simulink subsystem "StudentTemplate_MTMTAD006_M1"  (R2025a)
settings: Solver=VariableStepAuto  StartTime=0.0  StopTime=10.0  RelTol=1e-3
libraries: eeGeneralControl x3, simulink x2, slpidlib x1, cstblocks x1, dspstat3 x1
settings Model: Creator=JesseJabezArendse  LastModifiedBy=MTMTAD006

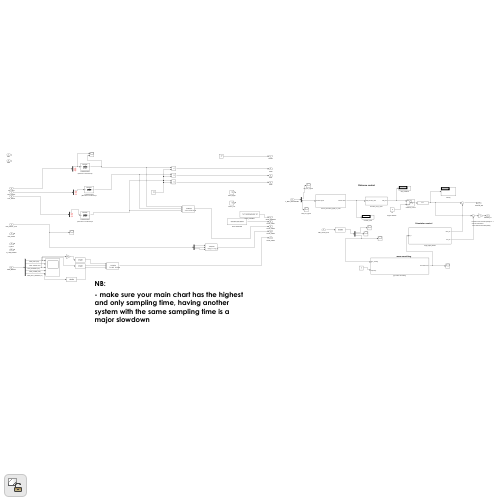
[thumbnail: Simulink's stored preview of the top-level diagram]
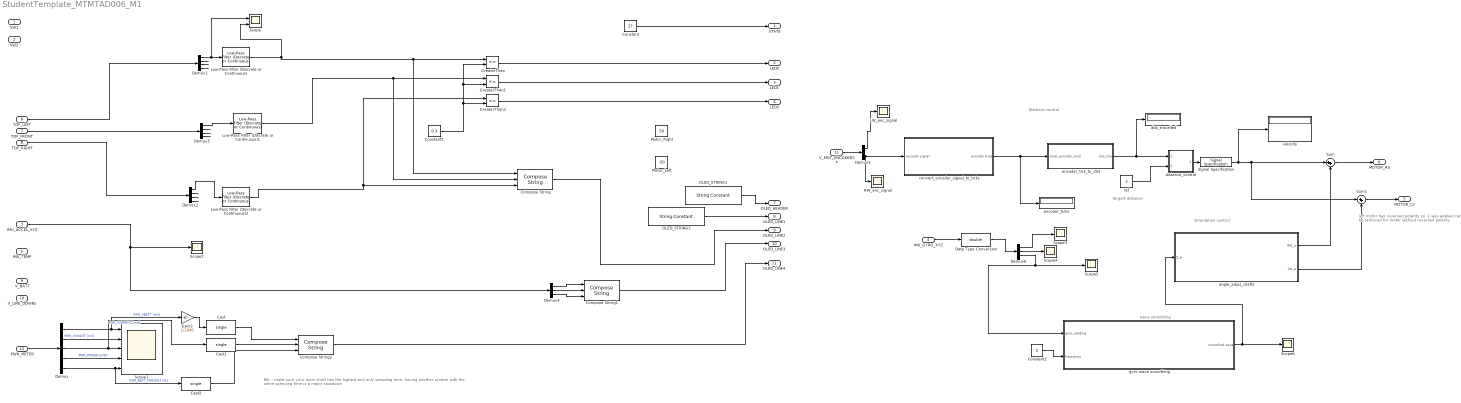
== system StudentTemplate_MTMTAD006_M1 ==
  note: left motor has reversed polarity so -1 was applied
      | can be removed for
      |  motor without reversed polarity
  note: targert distance
  note: wave smoothing
  note: Orientation control
  note: Distance control
  note: NB:
      |
      | - make sure your main chart has the highest and only sampling time, having another system with the same sampling time is a major slowdown
  SW1 : Inport
  SW2 : Inport  Port=2
  IMU_ACCEL_XYZ : Inport  Port=3
  IMU_GYRO_XYZ : Inport  Port=4
  IMU_TEMP : Inport  Port=5
  TOF_LEFT : Inport  Port=6
  TOF_FRONT : Inport  Port=7
  TOF_RIGHT : Inport  Port=8
  V_BATT : Inport  Port=9
  V_LINE_DOWNs : Inport  Port=10
  V_MOT_ENCODERSs : Inport  Port=11
  PWR_METER : Inport  Port=12
  Cast : DataTypeConversion  OutDataTypeStr=single  SaturateOnIntegerOverflow=off  RndMeth=Floor
  Cast1 : DataTypeConversion  OutDataTypeStr=single  SaturateOnIntegerOverflow=off  RndMeth=Floor
  Cast2 : DataTypeConversion  OutDataTypeStr=single  SaturateOnIntegerOverflow=off  RndMeth=Floor
  Compose String : ComposeString  Format="\"L%1.2f F%1.2f R%1.2f\""
  Compose String1 : ComposeString  Format="\"X%2.1f  Y%2.1f  Z%2.1f\""
  Compose String2 : ComposeString  Format="\"%1.2fV  %3.0fmA  %2.0f%%\""
  Constant : Constant  Value=27
  Constant1 : Constant  Value=0.3  SampleTime=-1
  Constant2 : Constant  Value=5
  Data Type Conversion : DataTypeConversion  OutDataTypeStr=double  SaturateOnIntegerOverflow=off  RndMeth=Floor
  Demux : Demux  Outputs=5
  Demux1 : Demux
  Demux2 : Demux
  Demux3 : Demux
  Demux4 : Demux  Outputs=3
  Demux5 : Demux  Outputs=2
  Demux6 : Demux  Outputs=3
  Gain2 : Gain  Gain=1/1000
  GreaterThan : RelationalOperator  Operator=<=  OutDataTypeStr=boolean  RndMeth=Simplest  InputSameDT=off
  GreaterThan1 : RelationalOperator  Operator=<=  OutDataTypeStr=boolean  RndMeth=Simplest  InputSameDT=off
  GreaterThan2 : RelationalOperator  Operator=<=  OutDataTypeStr=boolean  RndMeth=Simplest  InputSameDT=off
  LW_enc_signal : Scope
      settings: ActiveDisplayYMinimum=0.18771853517235504  ActiveDisplayYMaximum=0.24579643082508262  DataLoggingVariableName=ScopeData3
  Low-Pass Filter (Discrete or Continuous) : eeGeneralControl/Low-Pass Filter (Discrete or Continuous)  K=1  T=0.1  B=inf  A=-inf  init_option=Inherited from block input  x0=0  Ts=-1
  Low-Pass Filter (Discrete or Continuous)1 : eeGeneralControl/Low-Pass Filter (Discrete or Continuous)  K=1  T=0.1  B=inf  A=-inf  init_option=Inherited from block input  x0=0  Ts=-1
  Low-Pass Filter (Discrete or Continuous)2 : eeGeneralControl/Low-Pass Filter (Discrete or Continuous)  K=1  T=0.1  B=inf  A=-inf  init_option=Inherited from block input  x0=0  Ts=-1
  Motor_Left : Constant  Value=-50
  Motor_Right : Constant  Value=50
  OLED_STRING1 : StringConstant  String="\"UCT MICROMOUSE '25\""
  OLED_STRING2 : StringConstant  String="\"Simulink Data Demo\""
  RW_enc_signal : Scope
      settings: ActiveDisplayYMinimum=-0.18879534928548519  ActiveDisplayYMaximum=0.86303657781243615  DataLoggingVariableName=ScopeData4
  Scope : Scope  NumInputPorts=2
      settings: ActiveDisplayYMinimum=0.22759  ActiveDisplayYMaximum=0.52326  DataLoggingVariableName=ScopeData7
  Scope1 : Scope  NumInputPorts=5
      settings: ActiveDisplayYMinimum=-437.5  ActiveDisplayYMaximum=3937.5  DataLoggingVariableName=ScopeData6
  Scope{2..6} (5 alike) : Scope
      Scope2 settings: DataLoggingVariableName=ScopeData5
      Scope3 settings: ActiveDisplayYMinimum=-6.6655610351062915  ActiveDisplayYMaximum=8.47328179489563
      Scope4 settings: ActiveDisplayYMinimum=-9.9323014882304754  ActiveDisplayYMaximum=8.7797280520113681  DataLoggingVariableName=ScopeData10
      Scope5 settings: ActiveDisplayYMinimum=-4.0435245770175019  ActiveDisplayYMaximum=1.9742402712877856  DataLoggingVariableName=ScopeData9
      Scope6 settings: ActiveDisplayYMinimum=-2.7558239104233082  ActiveDisplayYMaximum=4.258969164786496  DataLoggingVariableName=ScopeData11
  Signal Specification : SignalSpecification  Dimensions=1
  Sum : Sum  Inputs=|++
  Sum1 : Sum  Inputs=|++
  angle_adjus_draft2 : Subsystem
  convert_encoder_signal_to_ticks : Subsystem
  dist_travelled : Display
  distance_control : Stateflow chart  TreatAsAtomicUnit=on
  encoder_tick_to_dist : Subsystem
  encoder_ticks : Display
  "gyro wave smoothing " : Subsystem
  ref : Constant  Value=2
  velocity : Display
  STATE : Outport
  LED0 : Outport  Port=2
  LED1 : Outport  Port=3
  LED2 : Outport  Port=4
  MOTOR_LS : Outport  Port=5
  MOTOR_RS : Outport  Port=6
  OLED_HEADER : Outport  Port=7
  OLED_LINE1 : Outport  Port=8
  OLED_LINE2 : Outport  Port=9
  OLED_LINE3 : Outport  Port=10
  OLED_LINE4 : Outport  Port=11
  wires:
  TOF_FRONT/1 -> Demux3/1
  OLED_STRING2/1 -> OLED_LINE1/1
  Demux2/1 -> Low-Pass Filter (Discrete or Continuous)2/1
  Demux2/3 -> ?
  Demux2/2 -> ?
  Demux2/4 -> ?
  Compose String1/1 -> OLED_LINE3/1
  Low-Pass Filter (Discrete or Continuous)1/1 -> Compose String/2, GreaterThan1/1
  GreaterThan1/1 -> LED1/1
  Demux3/3 -> ?
  TOF_RIGHT/1 -> Demux2/1
  Demux3/4 -> ?
  Demux3/2 -> ?
  Demux1/2 -> ?
  Demux3/1 -> Low-Pass Filter (Discrete or Continuous)1/1
  OLED_STRING1/1 -> OLED_HEADER/1
  Demux1/1 -> Scope/1, Low-Pass Filter (Discrete or Continuous)/1
  Compose String/1 -> OLED_LINE2/1
  Constant1/1 -> GreaterThan2/2, GreaterThan1/2, GreaterThan/2
  Demux1/4 -> ?
  GreaterThan2/1 -> LED2/1
  TOF_LEFT/1 -> Demux1/1
  GreaterThan/1 -> LED0/1
  Demux1/3 -> ?
  PWR_METER/1 -> Demux/1
  Demux/1 -> Scope1/1, Gain2/1  "PWR_VBATT [mV]"
  Demux/2 -> Scope1/2  "PWR_VSHUNT [mV]"
  Demux/3 -> Scope1/3, Cast1/1  "PWR_CURRENT [mA]"
  Demux/4 -> Scope1/4  "PWR_POWER [mW]"
  Demux/5 -> Scope1/5, Cast2/1  "PWR_BATT_PERCENT [%]"
  IMU_ACCEL_XYZ/1 -> Demux4/1, Scope2/1
  Demux4/1 -> Compose String1/1
  Demux4/2 -> Compose String1/2
  Demux4/3 -> Compose String1/3
  Compose String2/1 -> OLED_LINE4/1
  Gain2/1 -> Cast/1
  Cast/1 -> Compose String2/1
  Cast1/1 -> Compose String2/2
  Cast2/1 -> Compose String2/3
  Low-Pass Filter (Discrete or Continuous)2/1 -> Compose String/3, GreaterThan2/1
  Low-Pass Filter (Discrete or Continuous)/1 -> Scope/2, Compose String/1, GreaterThan/1
  Constant/1 -> STATE/1
  Demux5/2 -> convert_encoder_signal_to_ticks/1(encoder signal), RW_enc_signal/1
  Demux5/1 -> LW_enc_signal/1
  V_MOT_ENCODERSs/1 -> Demux5/1
  Signal Specification/1 -> Sum/1, Sum1/1, velocity/1
  distance_control/1(ang_vel) -> Signal Specification/1
  ref/1 -> distance_control/2(target)
  convert_encoder_signal_to_ticks/1(encoder ticks) -> encoder_tick_to_dist/1(total_encoder_ticks), encoder_ticks/1
  encoder_tick_to_dist/1(dist_trav) -> distance_control/1(dist_trav), dist_travelled/1
  Sum1/1 -> MOTOR_LS/1
  IMU_GYRO_XYZ/1 -> Data Type Conversion/1
  Demux6/1 -> Scope3/1
  Demux6/2 -> Scope4/1
  Sum/1 -> MOTOR_RS/1
  angle_adjus_draft2/1(RW_w) -> Sum/2
  angle_adjus_draft2/2(LW_w) -> Sum1/2
  Data Type Conversion/1 -> Demux6/1
  Demux6/3 -> Scope5/1, "gyro wave smoothing "/1(gyro_reading)
  Constant2/1 -> "gyro wave smoothing "/2(frequency)
  "gyro wave smoothing "/1(smoothed wave) -> angle_adjus_draft2/1(Z_w), Scope6/1

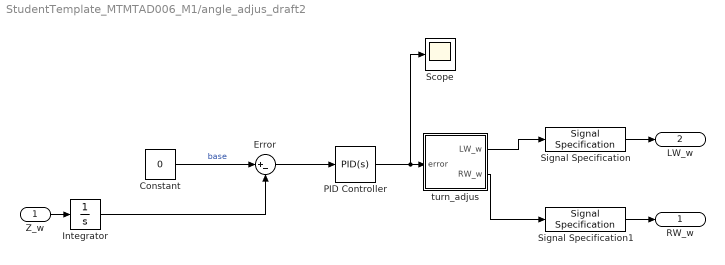
== system StudentTemplate_MTMTAD006_M1/angle_adjus_draft2 ==
  Z_w : Inport
  Constant : Constant  Value=0
  Error : Sum  Inputs=|+-
  Integrator : Integrator
  PID Controller : slpidlib/PID Controller  Controller=PID  Form=Parallel  TimeDomain=Continuous-time  UseExternalTs=off  SampleTime=-1  IntegratorMethod=Forward Euler  FilterMethod=Forward Euler  ControllerParametersSource=internal  P=3.2  I=1  UseKiTs=off  D=.001  UseExternalDerivativeSource=off  N=100  UseFilter=on  TunerSelectOption=Transfer Function Based (PID Tuner App)  InitialConditionSource=internal  InitialConditionForIntegrator=0  InitialConditionForFilter=0  DifferentiatorICPrevScaledInput=0  ExternalReset=none  TrackingMode=off  Kt=1  LimitOutput=off  SatLimitsSource=internal  UpperSaturationLimit=inf  LowerSaturationLimit=-inf  LinearizeAsGain=on  AntiWindupMode=none  Kb=1  LimitIntegrator=off  UpperIntegratorSaturationLimit=inf  LowerIntegratorSaturationLimit=-inf  POutMin=[]  POutMax=[]  IOutMin=[]  IOutMax=[]  DOutMin=[]  DOutMax=[]  NOutMin=[]  NOutMax=[]  SumOutMin=[]  SumOutMax=[]  SaturationOutMin=[]  SaturationOutMax=[]  PParamMin=[]  PParamMax=[]  IParamMin=[]  IParamMax=[]  DParamMin=[]  DParamMax=[]  NParamMin=[]  NParamMax=[]  KbParamMin=[]  KbParamMax=[]  KtParamMin=[]  KtParamMax=[]  KbOutMin=[]  KbOutMax=[]  KtOutMin=[]  KtOutMax=[]  IntegratorOutMin=[]  IntegratorOutMax=[]  FilterOutMin=[]  FilterOutMax=[]  SumI1OutMin=[]  SumI1OutMax=[]  SumI2OutMin=[]  SumI2OutMax=[]  SumI3OutMin=[]  SumI3OutMax=[]  SumI4OutMin=[]  SumI4OutMax=[]  SumDOutMin=[]  SumDOutMax=[]  DifferentiatorOutMin=[]  DifferentiatorOutMax=[]  FilterDiffOutCoefMin=[]  FilterDiffOutCoefMax=[]  ReciprocalOutMin=[]  ReciprocalOutMax=[]  SumDenOutMin=[]  SumDenOutMax=[]  SumNumOutMin=[]  SumNumOutMax=[]  DivideOutMin=[]  DivideOutMax=[]  UdiffTsProdOutMin=[]  UdiffTsProdOutMax=[]  NTsProdOutMin=[]  NTsProdOutMax=[]  UintegralTsProdOutMin=[]  UintegralTsProdOutMax=[]  UngainTsProdOutMin=[]  UngainTsProdOutMax=[]  ClampingZeroOutDataTypeStr=Inherit: Inherit via back propagation  ClampingZeroOutMin=[]  ClampingZeroOutMax=[]  FilterDenConstantOutDataTypeStr=Inherit: Inherit via back propagation  FilterDenConstantOutMin=[]  FilterDenConstantOutMax=[]  PCopyOutDataTypeStr=Inherit: Inherit via back propagation  PCopyOutMin=[]  PCopyOutMax=[]  NCopyOutDataTypeStr=Inherit: Inherit via back propagation  NCopyOutMin=[]  NCopyOutMax=[]  IntegratorContinuousStateAttributes=''  IntegratorStateMustResolveToSignalObject=off  IntegratorRTWStateStorageClass=Auto  FilterContinuousStateAttributes=''  FilterStateMustResolveToSignalObject=off  FilterRTWStateStorageClass=Auto  ParallelPVariant=InternalParameters  IdealPVariant=Disabled  IVariant=InternalParameters  DVariant=InternalParameters  IntegratorVariant=Continuous  SatVariant=Disabled  AWVariant=Passthrough  PCopyVariant=Disabled  TRVariant=Disabled  FdbkBlocksVariant=Forward  IdealPFdbkVariant=Disabled  SatFdbkVariant=Disabled  DerivativeFilterVariant=ContFilter  NVariant=InternalParameters  NCopyVariant=Disabled  FilterICVariant=InternalICsFilter  IntegratorICVariant=InternalICs  ExternalResetVariant=Disabled  TRSumVariant=Passthrough  SumFdbkVariant=Disabled  SumVariant=Sum_PID  TsampFilterVariant=InternalTs  TsampNgainVariant=Passthrough  TsampIntegralVariant=Disabled_SignalSpec  ExternalSaturationOutDataTypeStr=Inherit: Same as second input  DerivativeSourceVariant=ErrorSignal  PreIntVariant=InternalPreInt
  Scope : Scope
      settings: ActiveDisplayYMinimum=-1.13512117627545  ActiveDisplayYMaximum=1.044179082205777  DataLoggingVariableName=ScopeData8
  Signal Specification : SignalSpecification  Dimensions=1
  Signal Specification1 : SignalSpecification  Dimensions=1
  turn_adjus : Stateflow chart  TreatAsAtomicUnit=on
  RW_w : Outport
  LW_w : Outport  Port=2
  wires:
  Signal Specification1/1 -> RW_w/1
  Signal Specification/1 -> LW_w/1
  turn_adjus/2(RW_w) -> Signal Specification1/1
  turn_adjus/1(LW_w) -> Signal Specification/1
  PID Controller/1 -> turn_adjus/1(error), Scope/1
  Constant/1 -> Error/1  "base"
  Error/1 -> PID Controller/1
  Integrator/1 -> Error/2
  Z_w/1 -> Integrator/1

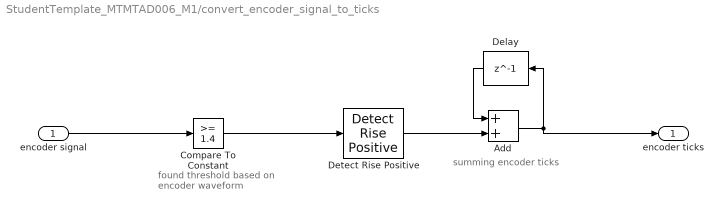
== system StudentTemplate_MTMTAD006_M1/convert_encoder_signal_to_ticks ==
  note: found threshold based
      |  on encoder waveform
  note: summing encoder ticks
  encoder signal : Inport
  Add : Sum
  Compare To Constant : simulink/Logic and Bit Operations/Compare To Constant  relop=>=  const=1.4  OutDataTypeStr=boolean
  Delay : Delay  DelayLength=1  InitialCondition=0
  Detect Rise Positive : simulink/Logic and Bit Operations/Detect Rise Positive  vinit=0  OutDataTypeStr=uint8
  encoder ticks : Outport
  wires:
  Delay/1 -> Add/1
  encoder signal/1 -> Compare To Constant/1
  Detect Rise Positive/1 -> Add/2
  Compare To Constant/1 -> Detect Rise Positive/1
  Add/1 -> Delay/1, encoder ticks/1

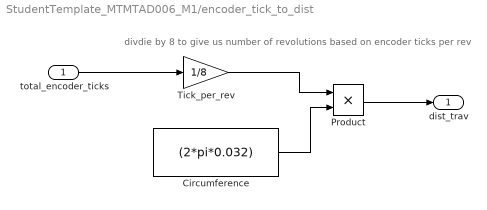
== system StudentTemplate_MTMTAD006_M1/encoder_tick_to_dist ==
  note: divdie by 8 to give us number of revolutions based on encoder ticks per rev
  total_encoder_ticks : Inport
  Circumference : Constant  Value=(2*pi*0.032)
  Product : Product
  Tick_per_rev : Gain  Gain=1/8
  dist_trav : Outport
  wires:
  total_encoder_ticks/1 -> Tick_per_rev/1
  Circumference/1 -> Product/2
  Tick_per_rev/1 -> Product/1
  Product/1 -> dist_trav/1

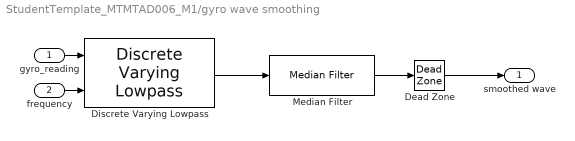
== system StudentTemplate_MTMTAD006_M1/gyro wave smoothing  ==
  gyro_reading : Inport
  frequency : Inport  Port=2
  Dead Zone : DeadZone
  Discrete Varying Lowpass : cstblocks/Linear Parameter Varying/Discrete Varying Lowpass  N=4  w0=0  Ts=0.01
  Median Filter : dspstat3/Median Filter  WindowLength=5  SimulateUsing=Interpreted execution
      settings: LibrarySourceBlock=|
      | dspfdesign/Median
      | Filter
  smoothed wave : Outport
  wires:
  gyro_reading/1 -> Discrete Varying Lowpass/1
  Dead Zone/1 -> smoothed wave/1
  frequency/1 -> Discrete Varying Lowpass/2
  Discrete Varying Lowpass/1 -> Median Filter/1
  Median Filter/1 -> Dead Zone/1

== stateflow chart StudentTemplate_MTMTAD006_M1/angle_adjus_draft2/turn_adjus ==
  state deafult
    during:
    LW_w = 0;
    RW_w = 0;
  state AdjustRight
    during:
    LW_w=error;
    RW_w = 0;
  state AdjustLeft
    during:
    RW_w = error;
    LW_w = 0;
  (default) -> deafult
  deafult -> AdjustRight [order 2] : [error>0]
  deafult -> AdjustLeft [order 1] : [error<0]
  data: error input; LW_w output; RW_w output

== stateflow chart StudentTemplate_MTMTAD006_M1/distance_control ==
  state Run
    during:
    ang_vel = 70;
  state Stop
    during:
    ang_vel =0;
  (default) -> Run
  Run -> Stop : [dist_trav>= target]
  data: dist_trav input; target input; ang_vel output
